simulink model "single_phase_ttype_inverter"  (R2026a)
settings: Solver=ode23tb  StopTime=simlength  FixedStep=tc  MaxStep=glb_time.tc
values from neighbouring files (symbols this model uses):
  afe_ctrl = param.afe.ctrl    [init_model.m]
  afe_pwm_phase_shift_mod1 = param.afe.behav.pwm_phase_shift_mod1    [init_model.m]
  DThs_init = param.thermal.DThs_init    [init_model.m]
  filters = param.ctrl.filters    [init_model.m]
  frt_data = param.frt.data    [init_model.m]
  glb_time = param.glb_time    [init_model.m]
  grid_emu = param.grid.emu    [init_model.m]
  kepsilon = param.spinv.kepsilon    [init_model.m]
  kp_align = param.ctrl.kp_align    [init_model.m]
  lim_down_align = param.ctrl.lim_down_align    [init_model.m]
  lim_up_align = param.ctrl.lim_up_align    [init_model.m]
  mavarage_filter_frequency_base_order = param.ctrl.mavarage_filter_frequency_base_order    [init_model.m]
  omega_set = param.spinv.omega_set    [init_model.m]
  single_phase_inverter_ctrl = param.spinv.ctrl    [init_model.m]
  Tambient = param.thermal.Tambient    [init_model.m]
  time_aux_power_supply_fault = param.sim.time_aux_power_supply_fault    [init_model.m]
  time_step_ref_1 = param.spinv.ref.time_step_ref_1    [init_model.m]
  time_step_ref_2 = param.spinv.ref.time_step_ref_2    [init_model.m]
  time_step_ref_3 = param.spinv.ref.time_step_ref_3    [init_model.m]
undefined symbols (not defined in the file or in its folder): delta_fht1, hwdata, ki_align, Ld_fht1, magnitude, omega_fht1, ts_inv, Vac_FS, Vdc_nom, Xbez
libraries: fl_lib x61, nesl_utility x39, moving_average_filter x11, moving_average_filter_cc x8, discrete_time_low_pass_filter x4, sl_discontinuities x3, single_phase_transformer_lib x3, linear_double_integrator_observer_ccaller x2, phase_shift_filter_ccaller x2, threephase_inductor_lib x1, dclink_for_two_levels x1, three_phase_pwm_modulator x1
(part 9 of 9)

== system single_phase_ttype_inverter/afe/AFE_control/afe_control/grid_voltage_phase_lock_loops/FHT-PLL/pll_stageA/filter_and_transformation/FHTalpha ==
  u : Inport
  Bus Selector : BusSelector  OutputSignals=output_pu_hat,output_pu_hat_dot
  C Caller : CCaller  FunctionName=first_harmonic_tracker_process_simulink  PortSpecificationStruct="%)30     .    B \\   8    (     @         %    \"     D    !     0         %  0 \"0    $    _    07)G3F%M90  4&]R=$YA;64 4V-O<&4     26YD97@     5'EP90      4VEZ90      27-';&]B86P   X    P    !@    @    $          4    (     0    ,    !         !   P!O=70 #@   #     &    \"     0         !0    @    !     P    $         $  # &]U=  .    .     8    (    !          %    \"     $    &     0         0  ...(+4988 chars)"
  Constant : Constant  Value=glb_time.ts_afe
  Constant1 : Constant  Value=12
  Constant4 : Constant  Value=afe_ctrl.fht_grid.omega_fht
  Constant5 : Constant  Value=afe_ctrl.fht_grid.delta_fht
  Constant6 : Constant  Value=afe_ctrl.fht_grid.Ld_fht(1)
  Constant7 : Constant  Value=afe_ctrl.fht_grid.Ld_fht(2)
  Data Type Conversion{1..2,6..9} (6 alike) : DataTypeConversion  OutDataTypeStr=single  SaturateOnIntegerOverflow=off  RndMeth=Floor
  Data Type Conversion10 : DataTypeConversion  OutDataTypeStr=double  SaturateOnIntegerOverflow=off  RndMeth=Floor
  Data Type Conversion3 : DataTypeConversion  OutDataTypeStr=uint8  SaturateOnIntegerOverflow=off  RndMeth=Floor
  Data Type Conversion4 : DataTypeConversion  OutDataTypeStr=double  SaturateOnIntegerOverflow=off  RndMeth=Floor
  Data Type Conversion5 : DataTypeConversion  OutDataTypeStr=uint8  SaturateOnIntegerOverflow=off  RndMeth=Floor
  Gain : Gain  Gain=1/afe_ctrl.fht_grid.omega_fht
  Step : Step  Time=0.0125  InitialValue=1  FinalValue=0
  ud_hat : Outport
  uq_hat : Outport  Port=2
  wires:
  Data Type Conversion9/1 -> C Caller/7
  Data Type Conversion8/1 -> C Caller/6
  Data Type Conversion7/1 -> C Caller/5
  Data Type Conversion6/1 -> C Caller/4
  Data Type Conversion5/1 -> C Caller/8
  Constant5/1 -> Data Type Conversion7/1
  Constant7/1 -> Data Type Conversion9/1
  Constant6/1 -> Data Type Conversion8/1
  Constant4/1 -> Data Type Conversion6/1
  Constant1/1 -> Data Type Conversion5/1
  Constant/1 -> Data Type Conversion1/1
  u/1 -> Data Type Conversion2/1
  Step/1 -> Data Type Conversion3/1
  Bus Selector/1 -> Data Type Conversion4/1  "<output_pu_hat>"
  C Caller/1 -> Bus Selector/1
  Data Type Conversion2/1 -> C Caller/2
  Data Type Conversion1/1 -> C Caller/3
  Data Type Conversion3/1 -> C Caller/1
  Data Type Conversion4/1 -> ud_hat/1
  Data Type Conversion10/1 -> Gain/1
  Bus Selector/2 -> Data Type Conversion10/1  "<output_pu_hat_dot>"
  Gain/1 -> uq_hat/1

== system single_phase_ttype_inverter/afe/AFE_control/afe_control/grid_voltage_phase_lock_loops/FHT-PLL/pll_stageA/filter_and_transformation/FHTbeta ==
  u : Inport
  Bus Selector : BusSelector  OutputSignals=output_pu_hat,output_pu_hat_dot
  C Caller : CCaller  FunctionName=first_harmonic_tracker_process_simulink  PortSpecificationStruct="%)30     .    B \\   8    (     @         %    \"     D    !     0         %  0 \"0    $    _    07)G3F%M90  4&]R=$YA;64 4V-O<&4     26YD97@     5'EP90      4VEZ90      27-';&]B86P   X    P    !@    @    $          4    (     0    ,    !         !   P!O=70 #@   #     &    \"     0         !0    @    !     P    $         $  # &]U=  .    .     8    (    !          %    \"     $    &     0         0  ...(+4988 chars)"
  Constant : Constant  Value=glb_time.ts_afe
  Constant1 : Constant  Value=14
  Constant4 : Constant  Value=afe_ctrl.fht_grid.omega_fht
  Constant5 : Constant  Value=afe_ctrl.fht_grid.delta_fht
  Constant6 : Constant  Value=afe_ctrl.fht_grid.Ld_fht(1)
  Constant7 : Constant  Value=afe_ctrl.fht_grid.Ld_fht(2)
  Data Type Conversion{1..2,6..9} (6 alike) : DataTypeConversion  OutDataTypeStr=single  SaturateOnIntegerOverflow=off  RndMeth=Floor
  Data Type Conversion10 : DataTypeConversion  OutDataTypeStr=double  SaturateOnIntegerOverflow=off  RndMeth=Floor
  Data Type Conversion3 : DataTypeConversion  OutDataTypeStr=uint8  SaturateOnIntegerOverflow=off  RndMeth=Floor
  Data Type Conversion4 : DataTypeConversion  OutDataTypeStr=double  SaturateOnIntegerOverflow=off  RndMeth=Floor
  Data Type Conversion5 : DataTypeConversion  OutDataTypeStr=uint8  SaturateOnIntegerOverflow=off  RndMeth=Floor
  Gain : Gain  Gain=1/afe_ctrl.fht_grid.omega_fht
  Step : Step  Time=0.0125  InitialValue=1  FinalValue=0
  ud_hat : Outport
  uq_hat : Outport  Port=2
  wires:
  Gain/1 -> uq_hat/1
  Bus Selector/2 -> Data Type Conversion10/1  "<output_pu_hat_dot>"
  Data Type Conversion10/1 -> Gain/1
  Data Type Conversion4/1 -> ud_hat/1
  Data Type Conversion3/1 -> C Caller/1
  Data Type Conversion1/1 -> C Caller/3
  Data Type Conversion2/1 -> C Caller/2
  C Caller/1 -> Bus Selector/1
  Bus Selector/1 -> Data Type Conversion4/1  "<output_pu_hat>"
  Step/1 -> Data Type Conversion3/1
  u/1 -> Data Type Conversion2/1
  Constant/1 -> Data Type Conversion1/1
  Constant1/1 -> Data Type Conversion5/1
  Constant4/1 -> Data Type Conversion6/1
  Constant6/1 -> Data Type Conversion8/1
  Constant7/1 -> Data Type Conversion9/1
  Constant5/1 -> Data Type Conversion7/1
  Data Type Conversion5/1 -> C Caller/8
  Data Type Conversion6/1 -> C Caller/4
  Data Type Conversion7/1 -> C Caller/5
  Data Type Conversion8/1 -> C Caller/6
  Data Type Conversion9/1 -> C Caller/7

== system single_phase_ttype_inverter/afe/AFE_control/afe_control/grid_voltage_phase_lock_loops/dq_pll/pll_stageA/sequences/alphabeta2xieta ==
  alpha : Inport
  beta : Inport  Port=2
  gamma : Inport  Port=3
  alphabeta2xieta_neg : MATLAB Function  TreatAsAtomicUnit=on
  alphabeta2xieta_pos : MATLAB Function  TreatAsAtomicUnit=on
  xi : Outport
  eta : Outport  Port=2
  Out3 : Outport  Port=3
  Out4 : Outport  Port=4
  wires:
  alpha/1 -> alphabeta2xieta_neg/1(alpha), alphabeta2xieta_pos/1(alpha)  "u_grid_alpha"
  beta/1 -> alphabeta2xieta_neg/2(beta), alphabeta2xieta_pos/2(beta)  "u_grid_beta"
  gamma/1 -> alphabeta2xieta_neg/3(gamma), alphabeta2xieta_pos/3(gamma)  "phase_grid"
  alphabeta2xieta_pos/1(xi) -> xi/1  "u_grid_pos_xi"
  alphabeta2xieta_pos/2(eta) -> eta/1  "u_grid_pos_eta"
  alphabeta2xieta_neg/1(xi) -> Out3/1  "u_grid_neg_xi"
  alphabeta2xieta_neg/2(eta) -> Out4/1  "u_grid_neg_eta"

== system single_phase_ttype_inverter/single_phase_inverter/single phase inverter control/single_phase_inverter_ctrl/single_phase_current_control/dqpi_current_controller/i2alphabeta/sogi/integrator_1 ==
  in : Inport
  Sum : Sum  Inputs=|++
  sample_time : Gain  Gain=glb_time.ts_inv
  unit_delay_1 : UnitDelay  SampleTime=-1
  out : Outport
  wires:
  in/1 -> sample_time/1
  sample_time/1 -> Sum/1
  Sum/1 -> unit_delay_1/1, out/1
  unit_delay_1/1 -> Sum/2

== system single_phase_ttype_inverter/single_phase_inverter/single phase inverter control/single_phase_inverter_ctrl/single_phase_current_control/dqpi_current_controller/i2alphabeta/sogi/integrator_2 ==
  in : Inport
  Sum : Sum  Inputs=|++
  sample_time : Gain  Gain=glb_time.ts_inv
  unit_delay_1 : UnitDelay  SampleTime=-1
  out : Outport
  wires:
  sample_time/1 -> Sum/1
  in/1 -> sample_time/1
  Sum/1 -> out/1, unit_delay_1/1
  unit_delay_1/1 -> Sum/2

== system single_phase_ttype_inverter/single_phase_inverter/single phase inverter control/single_phase_inverter_ctrl/single_phase_current_control/dqpi_current_controller/i2alphabeta/sogi_ccaller/Reset ==
  Step : Step  Time=0.025  InitialValue=1  FinalValue=0
  en : Outport
  wires:
  Step/1 -> en/1

== matlab function single_phase_ttype_inverter/single_phase_inverter/single phase inverter control/single_phase_inverter_ctrl/phase generator/bounder1 ==
  data: u input; y output
function y = bounder(u)
    
    y = -pi + mod(u+3*pi,2*pi);
   
end

== matlab function single_phase_ttype_inverter/afe/AFE_control/afe_control/grid_voltage_phase_lock_loops/FHT-PLL/pll_stageA/filter_and_transformation/abc2alphabeta ==
  data: a input; alpha output; b input; c input; beta output
function [alpha,beta] = abc2alphabeta(a,b,c)

alpha = 2/3*(a - 1/2*b - 1/2*c);
beta  = 1/sqrt(3)*(b - c);

end

== matlab function single_phase_ttype_inverter/afe/AFE_control/afe_control/grid_voltage_phase_lock_loops/FHT-PLL/pll_stageA/sequences/alphabeta2xieta ==
  data: alpha input; xi output; beta input; gamma input; eta output
function [xi,eta] = alphabeta2xieta_pos(alpha,beta,gamma)

    xi  =  (alpha*cos(gamma) + beta*sin(gamma));
    eta = (-alpha*sin(gamma) + beta*cos(gamma));

end

== matlab function single_phase_ttype_inverter/afe/AFE_control/afe_control/grid_voltage_phase_lock_loops/FHT-PLL/pll_stageB/bounder1 ==
  data: u input; y output
function y = bounder(u)
    y = -pi + mod(u+3*pi,2*pi);
end

== matlab function single_phase_ttype_inverter/afe/AFE_control/afe_control/FRT-VDE4110/FRT-Detection/LVRT_detector ==
  data: vxi_p input; vxi_n input; veta_n input; vxi_p_dot input; vxi_n_dot input; enable input; red_dyn_enabled input; pwr_lim_enable output; frt_exceeded output; reset input; frt_active output; frt_state output; red_dyn_active output
function [pwr_lim_enable, frt_exceeded, frt_active, frt_state, red_dyn_active]  = lvrt_detector(vxi_p,vxi_n,veta_n,vxi_p_dot,vxi_n_dot, enable, red_dyn_enabled, reset)

    persistent state count count2 state_pwr_lim
    
    LVRT_IDLE = 0;
    LVRT_ACTIVE = 1;
    LVRT_EXCEEDED = 2;
    
    PWR_LIM_DISABLED = 0;
    PWR_LIM_ENABLED  = 1;
    
    LVRT_VPOS_TH_LOW			= 0.85;
    LVRT_VPOS_TH_HIGH			= 1.15;
    LVRT_SEQ_DETECTION_HYST		= 0.1;
    LVRT_VNEG_TH				= 0.1;
    LVRT_VPOS_DOT_TH			= 2.0;
    LVRT_VNEG_DOT_TH			= 2.0;
    LVRT_VPOS_PWRLIM_TH			= 0.8;
    LVRT_VNEG_PWRLIM_TH			= 0.1;
    LVRT_PWRLIM_HYST			= 0.1;
    LVRT_VPOS_RED_DYN_TH        = 0.7;
    LVRT_VNEG_RED_DYN_TH        = 0.2;
    LVRT_TIME_HOLD_MAX          = 61000;
    
    RED_DYN_NOT_ACTIVE = 0;
    RED_DYN_ACTIVE     = 1;
        
    if isempty(state)
        state = LVRT_IDLE;
        state_pwr_lim = PWR_LIM_DISABLED;
        count = 0;
        count2 = 0;
    end

    vn = sqrt(vxi_n^2+veta_n^2);

    if enable == 1
        
        switch state
            
            case LVRT_IDLE
                if ((vxi_p > LVRT_VPOS_TH_HIGH || vxi_p < LVRT_VPOS_TH_LOW || vn > LVRT_VNEG_TH) ...
                     && (vxi_p_dot > LVRT_VPOS_DOT_TH || vxi_n_dot > LVRT_VNEG_DOT_TH) && ...
                     count2 > 1000)
                    state = LVRT_ACTIVE;
                end
                frt_active = 0;
                frt_exceeded = 0;
                count = 0;
                frt_state = LVRT_IDLE;
                state_pwr_lim = PWR_LIM_DISABLED;                  
                red_dyn_active = RED_DYN_NOT_ACTIVE;
                count2 = count2 + 1;

            case LVRT_ACTIVE
                count2 = 0;
                % LVRT condition not active anymore
                if (vxi_p >= LVRT_VPOS_TH_LOW  + LVRT_SEQ_DETECTION_HYST && ...
                    vxi_p <  LVRT_VPOS_TH_HIGH - LVRT_SEQ_DETECTION_HYST)
                    state = LVRT_IDLE;
                % LVRT exceeded
                elseif (count >= LVRT_TIME_HOLD_MAX)
                    state = LVRT_EXCEEDED;
                end
                
                % handle power limitation
                if (vxi_p < LVRT_VPOS_PWRLIM_TH || vn > LVRT_VNEG_PWRLIM_TH) 
                    state_pwr_lim = PWR_LIM_ENABLED;
                elseif (vxi_p > LVRT_VPOS_PWRLIM_TH + LVRT_PWRLIM_HYST && vn < LVRT_VPOS_PWRLIM_TH - LVRT_PWRLIM_HYST)
                    state_pwr_lim = PWR_LIM_DISABLED;                  
                end
                
                % handle reduced dynamic grid support
                if red_dyn_enabled && (vxi_p < LVRT_VPOS_RED_DYN_TH || vn > LVRT_VNEG_RED_DYN_TH)
                    red_dyn_active = RED_DYN_ACTIVE;
                else
                    red_dyn_active = RED_DYN_NOT_ACTIVE;
                end
                 
                frt_active = 1;
                frt_exceeded = 0;
                frt_state = LVRT_ACTIVE;
                
                count = count + 1;
            
            case LVRT_EXCEEDED

                if ((reset == 1) || (enable == 0))
                    state = LVRT_IDLE;
                else
                    state = LVRT_EXCEEDED;
                end
                
                frt_exceeded = 1;
                frt_active = 0; 
                frt_state = LVRT_EXCEEDED;
                red_dyn_active = RED_DYN_NOT_ACTIVE;
            
            otherwise
                state = LVRT_IDLE;
                frt_active = 0;
                frt_exceeded = 0;
                frt_state = LVRT_IDLE;
                red_dyn_active = RED_DYN_NOT_ACTIVE;
        end
        
        if state_pwr_lim == PWR_LIM_ENABLED
            pwr_lim_enable = 1;
        else
            pwr_lim_enable = 0;
        end      
    else
        state = LVRT_IDLE;
        frt_active = 0;
        pwr_lim_enable = 0;
        frt_exceeded = 0;
        frt_state = LVRT_IDLE;
        red_dyn_active = RED_DYN_NOT_ACTIVE;
    end
end

== matlab function single_phase_ttype_inverter/afe/AFE_control/afe_control/grid_voltage_phase_lock_loops/FHT-PLL/pll_stageB/double_integrator_observer/bounder1 ==
  data: u input; y output
function y = bounder(u)
    
    y = -pi + mod(u+3*pi,2*pi);
    
end

== matlab function single_phase_ttype_inverter/afe/AFE_control/afe_control/grid_voltage_phase_lock_loops/FHT-PLL/pll_stageB/double_integrator_observer/bounder2 ==
  data: u input; y output
function y = bounder(u)
    
    y = -pi + mod(u+3*pi,2*pi);
    
end

== matlab function single_phase_ttype_inverter/afe/AFE_control/afe_control/grid_voltage_phase_lock_loops/DDSRF-PLL/pll_stageA/filter_and_transformation/abc2alphabeta ==
  data: a input; alpha output; b input; c input; beta output
function [alpha,beta] = abc2alphabeta(a,b,c)

alpha = 2/3*(a - 1/2*b - 1/2*c);
beta  = 1/sqrt(3)*(b - c);

end

== matlab function single_phase_ttype_inverter/afe/AFE_control/afe_control/grid_voltage_phase_lock_loops/DDSRF-PLL/pll_stageA/sequences/ddsrf/alphabeta2xieta_neg ==
  data: alpha input; xi output; beta input; gamma input; eta output
function [xi,eta] = alphabeta2xieta_neg(alpha,beta,gamma)

    xi  = alpha*cos(gamma) - beta*sin(gamma);
    eta = alpha*sin(gamma) + beta*cos(gamma);

end

== matlab function single_phase_ttype_inverter/afe/AFE_control/afe_control/grid_voltage_phase_lock_loops/DDSRF-PLL/pll_stageB/double_integrator_observer/bounder1 ==
  data: u input; y output
function y = bounder(u)
    
    y = -pi + mod(u+3*pi,2*pi);
    
end

== matlab function single_phase_ttype_inverter/afe/AFE_control/afe_control/grid_voltage_phase_lock_loops/DDSRF-PLL/pll_stageB/double_integrator_observer/bounder2 ==
  data: u input; y output
function y = bounder(u)
    
    y = -pi + mod(u+3*pi,2*pi);
    
end

== matlab function single_phase_ttype_inverter/afe/AFE_control/afe_control/grid_voltage_phase_lock_loops/dq_pll/pll_stageB/double_integrator_observer/bounder1 ==
  data: u input; y output
function y = bounder(u)
    
    y = -pi + mod(u+3*pi,2*pi);
    
end

== matlab function single_phase_ttype_inverter/afe/AFE_control/afe_control/grid_voltage_phase_lock_loops/dq_pll/pll_stageA/mormalization_and_transformation/abc2alphabeta ==
  data: a input; alpha output; b input; c input; beta output
function [alpha,beta] = abc2alphabeta(a,b,c)

alpha = 2/3*(a - 1/2*b - 1/2*c);
beta  = 1/sqrt(3)*(b - c);

end

== matlab function single_phase_ttype_inverter/afe/AFE_control/afe_control/grid_voltage_phase_lock_loops/dq_pll/pll_stageA/sequences/alphabeta2xieta/alphabeta2xieta_neg ==
  data: alpha input; xi output; beta input; gamma input; eta output
function [xi,eta] = alphabeta2xieta_neg(alpha,beta,gamma)

    xi  = alpha*cos(gamma) - beta*sin(gamma);
    eta = alpha*sin(gamma) + beta*cos(gamma);

end

== matlab function single_phase_ttype_inverter/afe/AFE_control/afe_control/grid_voltage_phase_lock_loops/dq_pll/pll_stageA/sequences/alphabeta2xieta/alphabeta2xieta_pos ==
  data: alpha input; xi output; beta input; gamma input; eta output
function [xi,eta] = alphabeta2xieta_pos(alpha,beta,gamma)

    xi  =  alpha*cos(gamma) + beta*sin(gamma);
    eta = -alpha*sin(gamma) + beta*cos(gamma);

end

== matlab function single_phase_ttype_inverter/afe/AFE_control/afe_control/FRT-VDE4110/FRT-PosNegReactiveCurrentReferences/avg_flt_500ms/avg_flt_1 ==
  data: x input; y1 output; w input; ts input; enable input
function y1  = avg_flt(x,w,ts, enable)

    persistent x_int x_int_1 y_N N

    N = (1/(w/(2*pi)))/ts+1;

    if isempty(x_int)
        x_int_1 = 0;
        y_N = zeros(1,N);
        y1 = 0;
    end


    if enable == 1
        x_int = x * ts * w + x_int_1;
        x_int_1 = x_int;
        y_N(1,1) = x_int;
        y1 = 1/(2*pi)*((y_N(1,1) - y_N(1,N)));
        for i = 1:(N-1)
            y_N(1,N+1-i) = y_N(1,N-i); 
        end
    else
        y1 = 1/(2*pi)*((y_N(1,1) - y_N(1,N)));
    end
end

== matlab function single_phase_ttype_inverter/afe/AFE_control/afe_control/islanding_mode_detector/MATLAB Function ==
  data: alpha input; xi output; beta input; gamma input; eta output
function [xi,eta] = alphabeta2pos(alpha,beta,gamma)

    xi  =  alpha*cos(gamma) + beta*sin(gamma);
    eta = -alpha*sin(gamma) + beta*cos(gamma);

end

== matlab function single_phase_ttype_inverter/afe/AFE_control/afe_control/islanding_mode_detector/bounder ==
  data: u input; y output
function y = bounder(u)
    
    u = -pi + mod(u+3*pi,2*pi);
    
    y = u;
end

== matlab function single_phase_ttype_inverter/afe/AFE_control/afe_control/grid_voltage_phase_lock_loops/dq_pll/pll_stageB/double_integrator_observer/bounder2 ==
  data: u input; y output
function y = bounder(u)
    
    y = -pi + mod(u+3*pi,2*pi);
    
end

== matlab function single_phase_ttype_inverter/afe/AFE_control/afe_control/current_ctrl/inner_current_ctrl/anti_wind_up_ff/MATLAB Function1 ==
  data: da input; das output; db input; dc input; scaling input; dbs output; dcs output
function [das, dbs, dcs] = fcn(da,db,dc,scaling)

das = da/scaling;
dbs = db/scaling;
dcs = dc/scaling;

== matlab function single_phase_ttype_inverter/afe/AFE_control/afe_control/FRT-VDE4110/FRT-PosNegReactiveCurrentReferences/avg_flt_500ms1/avg_flt_1 ==
  data: x input; y1 output; w input; ts input; enable input
function y1  = avg_flt(x,w,ts, enable)

    persistent x_int x_int_1 y_N N

    N = (1/(w/(2*pi)))/ts+1;

    if isempty(x_int)
        x_int_1 = 0;
        y_N = zeros(1,N);
        y1 = 0;
    end


    if enable == 1
        x_int = x * ts * w + x_int_1;
        x_int_1 = x_int;
        y_N(1,1) = x_int;
        y1 = 1/(2*pi)*((y_N(1,1) - y_N(1,N)));
        for i = 1:(N-1)
            y_N(1,N+1-i) = y_N(1,N-i); 
        end
    else
        y1 = 1/(2*pi)*((y_N(1,1) - y_N(1,N)));
    end
end

== matlab function single_phase_ttype_inverter/afe/AFE_control/afe_control/FRT-VDE4110/FRT-PosNegReactiveCurrentReferences/avg_flt_500ms2/avg_flt_1 ==
  data: x input; y1 output; w input; ts input; enable input
function y1  = avg_flt(x,w,ts, enable)

    persistent x_int x_int_1 y_N N

    N = (1/(w/(2*pi)))/ts+1;

    if isempty(x_int)
        x_int_1 = 0;
        y_N = zeros(1,N);
        y1 = 0;
    end


    if enable == 1
        x_int = x * ts * w + x_int_1;
        x_int_1 = x_int;
        y_N(1,1) = x_int;
        y1 = 1/(2*pi)*((y_N(1,1) - y_N(1,N)));
        for i = 1:(N-1)
            y_N(1,N+1-i) = y_N(1,N-i); 
        end
    else
        y1 = 1/(2*pi)*((y_N(1,1) - y_N(1,N)));
    end
end

== matlab function single_phase_ttype_inverter/afe/AFE_control/afe_control/FRT-VDE4110/FRT-PosNegReactiveCurrentReferences/avg_flt_500ms3/avg_flt_1 ==
  data: x input; y1 output; w input; ts input; enable input
function y1  = avg_flt(x,w,ts, enable)

    persistent x_int x_int_1 y_N N

    N = (1/(w/(2*pi)))/ts+1;

    if isempty(x_int)
        x_int_1 = 0;
        y_N = zeros(1,N);
        y1 = 0;
    end


    if enable == 1
        x_int = x * ts * w + x_int_1;
        x_int_1 = x_int;
        y_N(1,1) = x_int;
        y1 = 1/(2*pi)*((y_N(1,1) - y_N(1,N)));
        for i = 1:(N-1)
            y_N(1,N+1-i) = y_N(1,N-i); 
        end
    else
        y1 = 1/(2*pi)*((y_N(1,1) - y_N(1,N)));
    end
end

== matlab function single_phase_ttype_inverter/afe/AFE_control/afe_control/grid_voltage_sequences/v_alphabeta2xieta/MATLAB Function ==
  data: alpha input; xi output; beta input; gamma input; eta output
function [xi,eta] = alphabeta2pos(alpha,beta,gamma)

    xi  =  alpha*cos(gamma) + beta*sin(gamma);
    eta = -alpha*sin(gamma) + beta*cos(gamma);

end

== matlab function single_phase_ttype_inverter/afe/AFE_control/afe_control/grid_voltage_sequences/v_alphabeta2xieta/MATLAB Function1 ==
  data: alpha input; xi output; beta input; gamma input; eta output
function [xi,eta] = alphabeta2neg(alpha,beta,gamma)

    xi  = alpha*cos(gamma) - beta*sin(gamma);
    eta = alpha*sin(gamma) + beta*cos(gamma);

end

== matlab function single_phase_ttype_inverter/afe/AFE_control/afe_control/grid_voltage_sequences/grid_voltage_sampling_and_alpha_beta_transformation/v_abc2alphabeta ==
  data: v_abc input; alpha output; beta output
function [alpha,beta] = abc2alphabeta(v_abc)

alpha = 2/3*(v_abc(1) - 1/2*v_abc(2) - 1/2*v_abc(3));
beta  = 1/sqrt(3)*(v_abc(2) - v_abc(3));

end

== matlab function single_phase_ttype_inverter/afe/AFE_control/afe_control/grid_current_sequences_and_reactive_pwr_ctrl/i_alphabeta2xieta/MATLAB Function ==
  data: alpha input; xi output; beta input; gamma input; eta output
function [xi,eta] = alphabeta2pos(alpha,beta,gamma)

    xi  =  alpha*cos(gamma) + beta*sin(gamma);
    eta = -alpha*sin(gamma) + beta*cos(gamma);

end

== matlab function single_phase_ttype_inverter/afe/AFE_control/afe_control/grid_current_sequences_and_reactive_pwr_ctrl/i_alphabeta2xieta/MATLAB Function1 ==
  data: alpha input; xi output; beta input; gamma input; eta output
function [xi,eta] = alphabeta2neg(alpha,beta,gamma)

    xi  = alpha*cos(gamma) - beta*sin(gamma);
    eta = alpha*sin(gamma) + beta*cos(gamma);

end

== matlab function single_phase_ttype_inverter/afe/AFE_control/afe_control/grid_current_sequences_and_reactive_pwr_ctrl/grid_current_sampling_and_alpha_beta_transformation/i_abc2alphabeta ==
  data: i_abc input; alpha output; beta output
function [alpha,beta] = abc2alphabeta(i_abc)

alpha = 2/3*(i_abc(1) - 1/2*i_abc(2) - 1/2*i_abc(3));
beta  = 1/sqrt(3)*(i_abc(2) - i_abc(3));

end

== matlab function single_phase_ttype_inverter/afe/AFE_control/afe_control/current_ctrl/inner_current_ctrl/anti_wind_up_ff/MATLAB Function ==
  data: a input; alpha output; b input; c input; beta output
function [alpha,beta] = abc2alphabeta(a,b,c)

alpha = 2/3*(a - 1/2*b - 1/2*c);
beta  = 1/sqrt(3)*(b - c);

end

== matlab function single_phase_ttype_inverter/afe/AFE_control/afe_control/current_ctrl/xieta2abc/MATLAB Function2 ==
  data: alpha input; a output; beta input; b output; c output
function [a,b,c] = alphabeta2abc(alpha,beta)

a = alpha;
b = -(1/2)*alpha + sqrt(3)/2*beta;
c = -(1/2)*alpha - sqrt(3)/2*beta;

end

== matlab function single_phase_ttype_inverter/afe/AFE_control/afe_control/current_ctrl/xieta2abc/Negative Sequence ==
  data: xi input; alpha output; eta input; phase input; beta output
function [alpha,beta] = neg2alphabeta(xi,eta,phase)

    alpha = xi*cos(phase)  + eta*sin(phase);
    beta  = -xi*sin(phase) + eta*cos(phase);

end

== matlab function single_phase_ttype_inverter/afe/AFE_control/afe_control/current_ctrl/xieta2abc/Positive Sequence ==
  data: xi input; alpha output; eta input; phase input; beta output
function [alpha,beta] = pos2alphabeta(xi,eta,phase)

    alpha = xi*cos(phase) - eta*sin(phase);
    beta  = xi*sin(phase) + eta*cos(phase);

end

== matlab function single_phase_ttype_inverter/afe/AFE_control/afe_control/grid_voltage_phase_lock_loops/dq_pll/pll_stageB/bounder1 ==
  data: u input; y output
function y = bounder(u)
    y = -pi + mod(u+3*pi,2*pi);
end

== matlab function single_phase_ttype_inverter/afe/AFE_control/afe_control/grid_voltage_phase_lock_loops/DDSRF-PLL/pll_stageA/sequences/ddsrf/alphabeta2xieta_neg1 ==
  data: alpha input; xi output; beta input; gamma input; eta output
function [xi,eta] = alphabeta2xieta_neg(alpha,beta,gamma)

    xi  = alpha*cos(gamma) - beta*sin(gamma);
    eta = alpha*sin(gamma) + beta*cos(gamma);

end

== matlab function single_phase_ttype_inverter/afe/AFE_control/afe_control/grid_voltage_phase_lock_loops/DDSRF-PLL/pll_stageA/sequences/ddsrf/alphabeta2xieta_pos ==
  data: alpha input; xi output; beta input; gamma input; eta output
function [xi,eta] = alphabeta2xieta_pos(alpha,beta,gamma)

    xi  =  alpha*cos(gamma) + beta*sin(gamma);
    eta = -alpha*sin(gamma) + beta*cos(gamma);

end

== matlab function single_phase_ttype_inverter/afe/AFE_control/afe_control/grid_voltage_phase_lock_loops/DDSRF-PLL/pll_stageA/sequences/ddsrf/alphabeta2xieta_pos1 ==
  data: alpha input; xi output; beta input; gamma input; eta output
function [xi,eta] = alphabeta2xieta_pos(alpha,beta,gamma)

    xi  =  alpha*cos(gamma) + beta*sin(gamma);
    eta = -alpha*sin(gamma) + beta*cos(gamma);

end

== matlab function single_phase_ttype_inverter/afe/AFE_control/afe_control/current_ctrl/current_transformation/alphabeta2xieta ==
  data: alpha input; xi output; beta input; gamma input; eta output
function [xi,eta] = alphabeta2xieta(alpha,beta,gamma)

    xi  =  alpha*cos(gamma) + beta*sin(gamma);
    eta = -alpha*sin(gamma) + beta*cos(gamma);

end

== matlab function single_phase_ttype_inverter/afe/AFE_control/afe_control/grid_voltage_phase_lock_loops/DDSRF-PLL/pll_stageA/sequences/ddsrf/bounder2 ==
  data: u input; y output
function y = bounder(u)
    
    y = -pi + mod(u+3*pi,2*pi);
    % y = mod(u, 2*pi);
    
end

== matlab function single_phase_ttype_inverter/afe/AFE_control/afe_control/grid_voltage_phase_lock_loops/DDSRF-PLL/pll_stageB/bounder1 ==
  data: u input; y output
function y = bounder(u)
    y = -pi + mod(u+3*pi,2*pi);
end

== matlab function single_phase_ttype_inverter/afe/brake/MATLAB Function ==
  data: u input; y output; udc_ref input
function y = fcn(u,udc_ref)

persistent enable_brake

udc_brake_min = 1.15;
udc_brake_max = 1.175;

if isempty(enable_brake)
    enable_brake = 0
end

if u >= udc_ref*udc_brake_max
    y = 15;
    enable_brake = 1;
elseif (u < udc_ref*udc_brake_max && u >= udc_ref*udc_brake_min && enable_brake == 1)
    y = 15;
    enable_brake = 1;
elseif (u < udc_ref*udc_brake_max && u >= udc_ref*udc_brake_min && enable_brake == 0)
    y = 0;
    enable_brake = 0;
else
    y = 0;
    enable_brake = 0;
end

% function y = fcn(u,udc_ref)
% 
% persistent enable_brake
% 
% udc_brake_min = 1.145;
% udc_brake_max = 1.165;
% 
% if isempty(enable_brake)
%     enable_brake = 0
% end
% 
% if u >= udc_ref*udc_brake_max
%     y = 15;
%     enable_brake = 1;
% elseif (u < udc_ref*udc_brake_max && u >= udc_ref*udc_brake_min && enable_brake == 1)
%     y = 15;
%     enable_brake = 1;
% elseif (u < udc_ref*udc_brake_max && u >= udc_ref*udc_brake_min && enable_brake == 0)
%     y = 0;
%     enable_brake = 0;
% else
%     y = 0;
%     enable_brake = 0;
end

== matlab function single_phase_ttype_inverter/single_phase_inverter/single phase inverter control/single_phase_inverter_ctrl/impedance_measure/Subsystem/MATLAB Function ==
  data: u input; y output; Vdc_FS input; Vac_FS input; Xbez input
function y = scaling(u, Vdc_FS, Vac_FS, Xbez)

y = Vdc_FS/Vac_FS*Xbez * u;

== matlab function single_phase_ttype_inverter/afe/AFE_control/afe_control/current_ctrl/current_transformation/uvw2alphabeta ==
  data: u input; alpha output; v input; w input; beta output
function [alpha,beta] = uvw2alphabeta(u,v,w)

alpha = 2/3*(u - 1/2*v - 1/2*w);
beta  = 2/3*(sqrt(3)/2*(v - w));

end

== matlab function single_phase_ttype_inverter/single_phase_inverter/single phase inverter control/single_phase_inverter_ctrl/sistem_identification/open loop u//f/dq2alphabeta/MATLAB Function ==
  data: d input; alpha output; q input; phase input; beta output
function [alpha, beta] = dq2alphabeta(d, q, phase)

alpha = d*cos(phase) - q*sin(phase);
beta = d*sin(phase) + q*cos(phase);

== matlab function single_phase_ttype_inverter/single_phase_inverter/single phase inverter control/single_phase_inverter_ctrl/single_phase_current_control/dqpi_current_controller/alphabeta2dq/MATLAB Function ==
  data: alpha input; d output; beta input; phase input; q output
function [d, q] = alphabeta2dq(alpha, beta, phase)

d = alpha*cos(phase) + beta*sin(phase);
q = -alpha*sin(phase) + beta*cos(phase);

== matlab function single_phase_ttype_inverter/single_phase_inverter/single phase inverter control/single_phase_inverter_ctrl/single_phase_current_control/dqpi_current_controller/dq2alphabeta/MATLAB Function ==
  data: d input; alpha output; q input; phase input; beta output
function [alpha, beta] = dq2alphabeta(d, q, phase)

alpha = d*cos(phase) - q*sin(phase);
beta = d*sin(phase) + q*cos(phase);
